simulink model "hydel"  (R2024b)
settings: Solver=VariableStepAuto  StartTime=0.0  StopTime=5  RelTol=1e-3
undefined symbols (not defined in the file): D1, Delta
libraries: spsThreePhaseTransformerTwoWindingsLib x1, spsSynchronousMachinepuStandardLib x1, spsVoltageMeasurementLib x1, spsThreePhaseSourceLib x1, spsThreePhaseParallelRLCLoadLib x1, spsHydraulicTurbineandGovernorLib x1, spsExcitationSystemLib x1, spsGroundLib x1, sps_lib x1
settings Model: Creator=Mahesh  LastModifiedBy=Mahesh

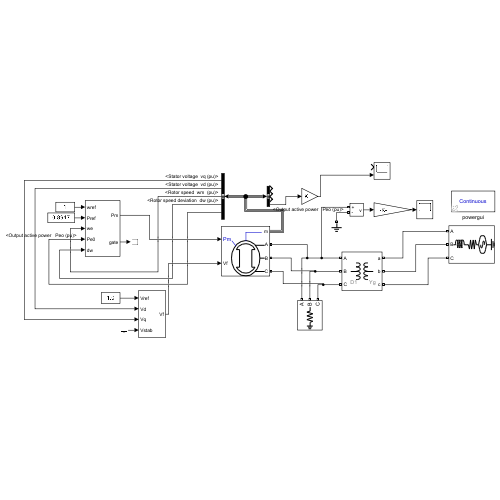
[thumbnail: Simulink's stored preview of the top-level diagram]
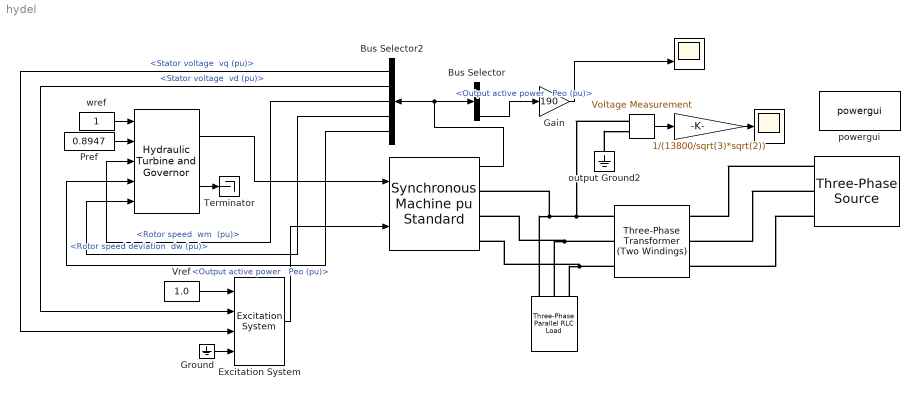
== system hydel ==
  "  " : spsThreePhaseTransformerTwoWindingsLib/Three-Phase Transformer (Two Windings)  Winding1Connection=Delta (D1)  Winding2Connection=Yg  CoreType=Three single-phase transformers  SetSaturation=off  Hysteresis=off  DataFile='hysteresis'  SetInitialFlux=off  Measurements=None  UNITS=pu  NominalPower=[ 210e6 60 ]  Winding1="[ 13.8e3 0.0027  0.08]"  Winding2=[ 230e3 0.0027 0.08]  Rm=500  Lm=500  L0=0.5  Saturation="[ 0,0  ;  0.005,1.2  ;  1.0,1.4 ]"  InitialFluxes=[ 0.8 , -0.8 , 0.7 ]  BreakLoop=off  DiscreteSolver=Trapezoidal iterative  DataType=off  TransfoNumber=0
  "   " : Gain  Gain=1/(13800/sqrt(3)*sqrt(2))  SaturateOnIntegerOverflow=on  OutDataTypeStr=Inherit: Same as input  ParamDataTypeStr=Inherit: Same as input
  "    " : spsSynchronousMachinepuStandardLib/Synchronous Machine pu Standard  PresetModel=No  MechanicalLoad=Mechanical power Pm  ShowDetailedParameters=on  RotorType=Salient-pole  Units=per unit standard parameters  MeasurementBus=off  NominalParameters="[ 190E6  13800   60 ]"  Reactances1=[ 31 32 33 34 35 36 37 ]  Reactances2=[ 1.305, 0.296, 0.252, 0.474, 0.243, 0.18 ]  dAxisTimeConstants=Short-circuit  qAxisTimeConstants=Open-circuit  TimeConstants1=[]  TimeConstants2=[]  TimeConstants3=[]  TimeConstants4=[]  TimeConstants5=[ 1.01, 0.053, 0.1 ]  TimeConstants6=[]  TimeConstants7=[]  TimeConstants8=[]  StatorResistance=2.8544e-3  Mechanical="[ 3.2 0  32]"  PolePairs=32  InitialConditions=[0 0 0 0 0 0 0 0 1]  SetSaturation=off  Saturation=[0.6404,0.7127,0.8441,0.9214,0.9956,1.082,1.19,1.316,1.457;0.7,0.7698,0.8872,0.9466,0.9969,1.046,1.1,1.151,1.201]  LoadFlowParameters=[1 150000000 0 0]  TsPowergui=0  TsBlock=-1  IterativeModel=Forward Euler  IterativeDiscreteModel=Trapezoidal non iterative  BusType=PV  Pref=0  Qref=0  Qmin=-inf  Qmax=inf  PLF=0  QLF=0
  "     " : spsVoltageMeasurementLib/Voltage Measurement  Tag=PoWeRsYsTeMmEaSuReMeNt  PhasorSimulation=off  OutputType=Magnitude  PSBequivalent=0
  "       " : spsThreePhaseSourceLib/Three-Phase Source  InternalConnection=Yg  VoltagePhases=off  Voltage=230e3  PhaseAngle=0  Voltage_phases=[25e3 25e3 25e3]/sqrt(3)  PhaseAngles_phases=[0 -120 +120]  Frequency=50  NonIdealSource=on  SpecifyImpedance=on  Resistance=0.529  Inductance=0.0140  ShortCircuitLevel=10000e6  BaseVoltage=230e3  XRratio=10  BusType=swing  Pref=10e3  Qref=0  Prefabc=[10e3, 10e3, 10e3]  Qrefabc=[0, 0, 0]  Qmin=-inf  Qmax=inf
  "                  " : spsThreePhaseParallelRLCLoadLib/Three-Phase Parallel RLC Load  LConnTagsString=A|B|C  Configuration=Y (grounded)  NominalVoltage=13.8e3  Vabc=[1e3 1e3 1e3]  Vabcp=[1e3 1e3 1e3]  NominalFrequency=60  UnbalancedPower=off  ActivePower=100e6  InductivePower=0  CapacitivePower=0  Pabc=[10e3 9e3 11e3]  QLabc=[100 90 110]  QCabc=[100 90 110]  Pabcp=[10e3 9e3 11e3]  QLabcp=[100 90 110]  QCabcp=[100 90 110]  Measurements=None  LoadType=constant Z
  "                         " : spsHydraulicTurbineandGovernorLib/Hydraulic Turbine and Governor  sm="[ 10/3  0.07 ]"  gate="[  0.01  0.97518  -0.1  0.1 ]"  reg="[  0.05  1.163  0.105  0  0.01  ]"  hyd="[  0  2.67  ]"  dref=0  po=1
  "                                       " : Scope
  "                                                                                 " : Scope  NumInputPorts=2
  Bus Selector : BusSelector  OutputSignals="Stator current,dq0 components.Stator voltage  vq (pu),dq0 components.Stator voltage  vd (pu),Output active power   Peo (pu)"
  Bus Selector2 : BusSelector  OutputSignals="dq0 components.Stator voltage  vq (pu),dq0 components.Stator voltage  vd (pu),Mechanical.Rotor speed  wm  (pu),Mechanical.Rotor speed deviation  dw (pu),Output active power   Peo (pu)"
  Excitation System : spsExcitationSystemLib/Excitation System  tr=20e-3  reg=[ 300, 0.001 ]  exc=[ 1, 0 ]  tgr=[ 0, 0 ]  damp=[ 0.01, 0.1 ]  sat=[ 0, 0 ]  lim=[ -11.5, 11.5, 0 ]  v0=[1,1.0]
  Gain : Gain  Gain=190
  Ground : Ground
  Pref : Constant  Value=0.8947
  Terminator : Terminator
  Vref : Constant  Value=1.0
  output Ground2 : spsGroundLib/Ground  LConnTagsString=a
  powergui : sps_lib/powergui  Priority=1  SimulationMode=Continuous  SampleTime=50e-6  frequency=60  Iterations=50  frequencyindice=60  Pbase=100e6  ErrMax=1e-4  UnitsV=kV  UnitsW=MW  buscounter=0  FunctionMessages=off  echomessages=off  EnableUseOfTLC=off  CurrentSourceSwitches=off  DisableSnubberDevices=off  DisableRonSwitches=off  DisableVfSwitches=off  DisplayEquations=off  AutomaticDiscreteSolvers=off  SolverType=Tustin/Backward Euler (TBE)  Interpol=off  ExternalGateDelay=off  methode=off  Ts=100  x0status=blocks  SPID=on  SwTol=0  HookPort=off  NonlinearTolerance=1e-4  nMaxIteration=100  ContinueOnMaxIteration=off  RestoreLinks=warning  ResistiveCurrentMeasurement=off  Frange=[0:2:500]  Ylog=off  Xlog=on  ShowGrid=off  save=off  variable=ZData  structure=0  ZoomFFT=off  StartTime=0.0  cycles=1  DisplayStyle=1  fundamental=60  FreqAxis=off  MaxFrequency=1000  frequencyindicesteady=1  RmsSteady=1  display=off
  wref : Constant
  wires:
  "     "/1 -> "   "/1
  "   "/1 -> "                                       "/1
  wref/1 -> "                         "/1
  Pref/1 -> "                         "/2
  Vref/1 -> Excitation System/1
  Ground/1 -> Excitation System/4
  "                         "/1 -> "    "/1
  "                         "/2 -> Terminator/1
  "    "/1 -> Bus Selector2/1, Bus Selector/1
  Bus Selector2/1 -> Excitation System/3  "<Stator voltage  vq (pu)>"
  Bus Selector2/2 -> Excitation System/2  "<Stator voltage  vd (pu)>"
  Bus Selector2/3 -> "                         "/3  "<Rotor speed  wm  (pu)>"
  Bus Selector2/5 -> "                         "/4  "<Output active power   Peo (pu)>"
  Bus Selector2/4 -> "                         "/5  "<Rotor speed deviation  dw (pu)>"
  Excitation System/1 -> "    "/2
  Bus Selector/4 -> Gain/1  "<Output active power   Peo (pu)>"
  Gain/1 -> "                                                                                 "/2
  connections:
  "  "/LConn1 -- "     "/LConn1 -- "                  "/LConn1 -- "    "/RConn1
  "  "/LConn2 -- "                  "/LConn2 -- "    "/RConn2
  "  "/LConn3 -- "                  "/LConn3 -- "    "/RConn3
  "       "/RConn1 -- "  "/RConn1
  "       "/RConn2 -- "  "/RConn2
  "       "/RConn3 -- "  "/RConn3
  output Ground2/LConn1 -- "     "/LConn2
